simulink subsystem "SRPTorque"  (R2024b)
settings: Solver=VariableStepAuto  StartTime=0.0  StopTime=10.0  RelTol=1e-3
undefined symbols (not defined in the file): spacecraft
libraries: sadlib x2
settings Model: Creator=marco  LastModifiedBy=ferru

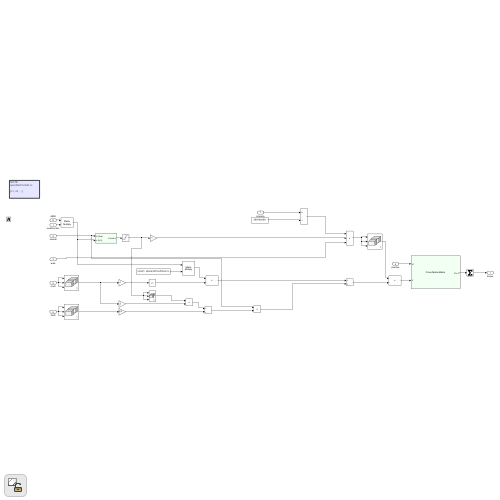
[thumbnail: Simulink's stored preview of the top-level diagram]
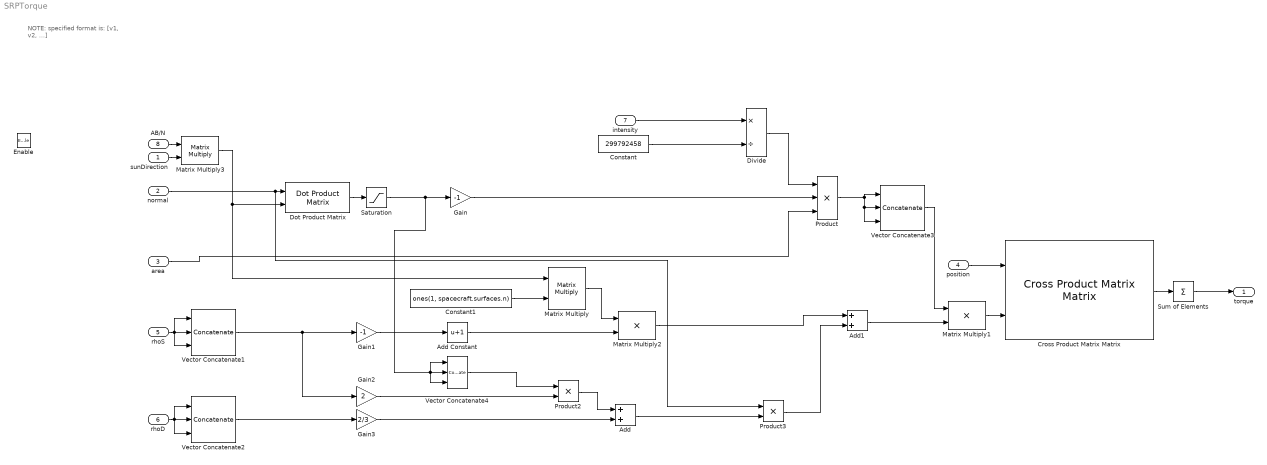
== system SRPTorque ==
  note: NOTE:
      | specified format is:
      |
      | [v1, v2, ...]
  sunDirection : Inport
  normal : Inport  Port=2
  area : Inport  Port=3
  position : Inport  Port=4
  rhoS : Inport  Port=5
  rhoD : Inport  Port=6
  intensity : Inport  Port=7
  AB/N : Inport  Port=8
  Enable : EnablePort  StatesWhenEnabling=reset
  Add : Sum
  Add Constant : Bias  Bias=1  SaturateOnIntegerOverflow=off
  Add1 : Sum
  Constant : Constant  Value=299792458
  Constant1 : Constant  Value=ones(1, spacecraft.surfaces.n)  VectorParams1D=off
  Cross Product Matrix Matrix : sadlib/Cross Product Matrix Matrix
      settings: SourceProductName=SAD Library
  Divide : Product  Inputs=*/
  "Dot Product Matrix " : sadlib/Dot Product Matrix   SystemSampleTime=-1  VariantActivationTime=update diagram  AllowFlexibleInterface=on  Latency=0  AutoFrameSizeCalculation=off
  Gain : Gain  Gain=-1
  Gain1 : Gain  Gain=-1
  Gain2 : Gain  Gain=2
  Gain3 : Gain  Gain=2/3
  Matrix Multiply : Product  Multiplication=Matrix(*)
  Matrix Multiply1 : Product
  Matrix Multiply2 : Product
  Matrix Multiply3 : Product  Multiplication=Matrix(*)
  Product : Product  Inputs=3
  Product2 : Product
  Product3 : Product
  Saturation : Saturate  UpperLimit=inf  LowerLimit=0
  Sum of Elements : Sum  Inputs=+  CollapseMode=Specified dimension  CollapseDim=2
  Vector Concatenate{1..4} (4 alike) : Concatenate  NumInputs=3  Mode=Multidimensional array
  torque : Outport  PortDimensions=[3, 1]
  wires:
  Matrix Multiply3/1 -> "Dot Product Matrix "/2, Matrix Multiply/1
  Constant/1 -> Divide/2
  normal/1 -> "Dot Product Matrix "/1, Product3/1
  Gain/1 -> Product/2
  Divide/1 -> Product/1
  area/1 -> Product/3
  Vector Concatenate1/1 -> Gain1/1, Gain2/1
  Gain1/1 -> Add Constant/1
  Add Constant/1 -> Matrix Multiply2/2
  Gain2/1 -> Product2/2
  Product2/1 -> Add/1
  Gain3/1 -> Add/2
  Add/1 -> Product3/2
  Product3/1 -> Add1/2
  position/1 -> Cross Product Matrix Matrix/1
  Cross Product Matrix Matrix/1 -> Sum of Elements/1
  Sum of Elements/1 -> torque/1
  intensity/1 -> Divide/1
  Matrix Multiply2/1 -> Add1/1
  Add1/1 -> Matrix Multiply1/2
  Matrix Multiply1/1 -> Cross Product Matrix Matrix/2
  rhoS/1 -> Vector Concatenate1/2, Vector Concatenate1/3, Vector Concatenate1/1
  rhoD/1 -> Vector Concatenate2/3, Vector Concatenate2/2, Vector Concatenate2/1
  Vector Concatenate2/1 -> Gain3/1
  Product/1 -> Vector Concatenate3/1, Vector Concatenate3/3, Vector Concatenate3/2
  Vector Concatenate3/1 -> Matrix Multiply1/1
  Constant1/1 -> Matrix Multiply/2
  Matrix Multiply/1 -> Matrix Multiply2/1
  Vector Concatenate4/1 -> Product2/1
  Saturation/1 -> Gain/1, Vector Concatenate4/2, Vector Concatenate4/3, Vector Concatenate4/1
  "Dot Product Matrix "/1 -> Saturation/1
  AB/N/1 -> Matrix Multiply3/1
  sunDirection/1 -> Matrix Multiply3/2
